simulink model "Presentation"  (Simulink 8.2)
settings: Solver=ode45  StartTime=0.0  StopTime=10.0  RelTol=1e-3
libraries: fuzblock x1
settings Model: Creator=hopefully  LastModifiedBy=hopefully
settings DataIOCC: SignalLoggingSaveFormat=Dataset
settings OptimizationCC: ExpressionDepthLimit=128
settings DebuggingCC: FcnCallInpInsideContextMsg=EnableAllAsError  StateNameClashWarn=none
settings GRTTargetCC: CombineOutputUpdateFcns=on  GRTInterface=off

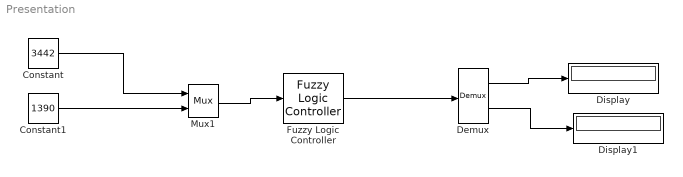
== system Presentation ==
  Constant : Constant  Value=3442
  Constant1 : Constant  Value=1390
  Demux : Demux  Outputs=2
  Display : Display
  Display1 : Display
  Fuzzy Logic Controller : fuzblock/Fuzzy Logic  Controller  fis=fismat
  Mux1 : Mux  Inputs=2
  wires:
  Mux1/1 -> Fuzzy Logic Controller/1
  Fuzzy Logic Controller/1 -> Demux/1
  Constant/1 -> Mux1/1
  Constant1/1 -> Mux1/2
  Demux/2 -> Display1/1
  Demux/1 -> Display/1
